simulink model "practica4"  (R2020b)
settings: Solver=ode15s  StartTime=0.0  StopTime=10.0  MaxStep=1E-2  RelTol=1e-3
libraries: fl_lib x10, nesl_utility x6, ee_lib x4, pid_lib x1
settings Model: Creator=demil  LastModifiedBy=demil
settings SolverCC: AlgebraicLoopSolver=LineSearch
settings DataIOCC: SaveFormat=Array  SaveOutput=off  SignalLogging=off  DSMLogging=off  ReturnWorkspaceOutputs=off  TimeSaveName=t
settings DebuggingCC: AlgebraicLoopMsg=none  ArtificialAlgebraicLoopMsg=none  MaxConsecutiveZCsMsg=none  ModelReferenceExtraNoncontSigs=none  OperatingPointInterfaceChecksumMismatchMsg=none

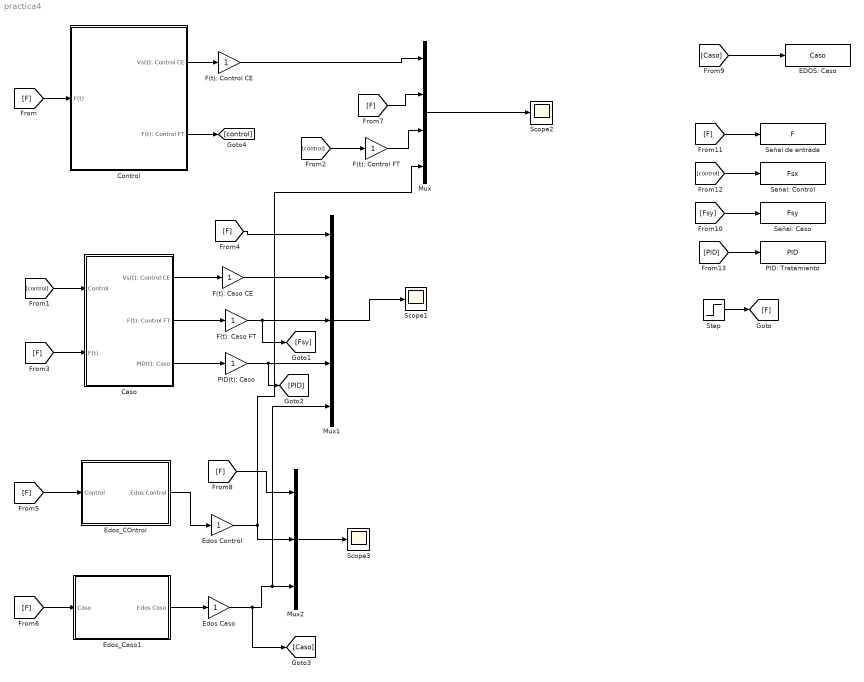
== system practica4 ==
  Caso : Subsystem
  Control : Subsystem
  EDOS: Caso : ToWorkspace  VariableName=Caso  SampleTime=-1
  Edos Caso : Gain
  Edos Control : Gain
  Edos_COntrol : Subsystem
  Edos_Caso1 : Subsystem
  F(t): Caso CE : Gain
  F(t): Caso FT : Gain
  F(t): Control CE : Gain
  F(t): Control FT : Gain
  Mux : Mux
  Mux1 : Mux  Inputs=5
  Mux2 : Mux  Inputs=3
  PID(t): Caso : Gain
  PID: Tratamiento : ToWorkspace  VariableName=PID  SampleTime=-1
  Scope1 : Scope
  Scope2 : Scope
  Scope3 : Scope
  Señal de entrada : ToWorkspace  VariableName=F  SampleTime=-1
  Señal: Caso : ToWorkspace  VariableName=Fsy  SampleTime=-1
  Señal: Control : ToWorkspace  VariableName=Fsx  SampleTime=-1
  Step : Step  Time=0  SampleTime=0
  wires:
  [PID] -> PID: Tratamiento/1
  PID(t): Caso/1 -> Mux1/4, [PID]
  [Fsy] -> Señal: Caso/1
  [control] -> F(t): Control FT/1
  [F] -> Señal de entrada/1
  [F] -> Caso/2(F(t))
  [F] -> Mux1/1
  Mux/1 -> Scope2/1
  F(t): Caso FT/1 -> [Fsy], Mux1/3
  Step/1 -> [F]
  F(t): Caso CE/1 -> Mux1/2
  Control/1(Vs(t): Control CE) -> F(t): Control CE/1
  Mux1/1 -> Scope1/1
  Caso/3(PID(t): Caso) -> PID(t): Caso/1
  [control] -> Caso/1(Control)
  F(t): Control FT/1 -> Mux/3
  [control] -> Señal: Control/1
  [F] -> Control/1(F(t))
  Control/2(F(t): Control FT) -> [control]
  F(t): Control CE/1 -> Mux/1
  Caso/1(Vs(t): Control CE) -> F(t): Caso CE/1
  Caso/2(F(t): Control FT) -> F(t): Caso FT/1
  [F] -> Edos_COntrol/1(Control)
  Edos_COntrol/1(Edos Control) -> Edos Control/1
  Mux2/1 -> Scope3/1
  [F] -> Edos_Caso1/1(Caso)
  Edos_Caso1/1(Edos Caso) -> Edos Caso/1
  Edos Caso/1 -> [Caso], Mux1/5, Mux2/3
  Edos Control/1 -> Mux/4, Mux2/2
  [F] -> Mux2/1
  [F] -> Mux/2
  [Caso] -> EDOS: Caso/1

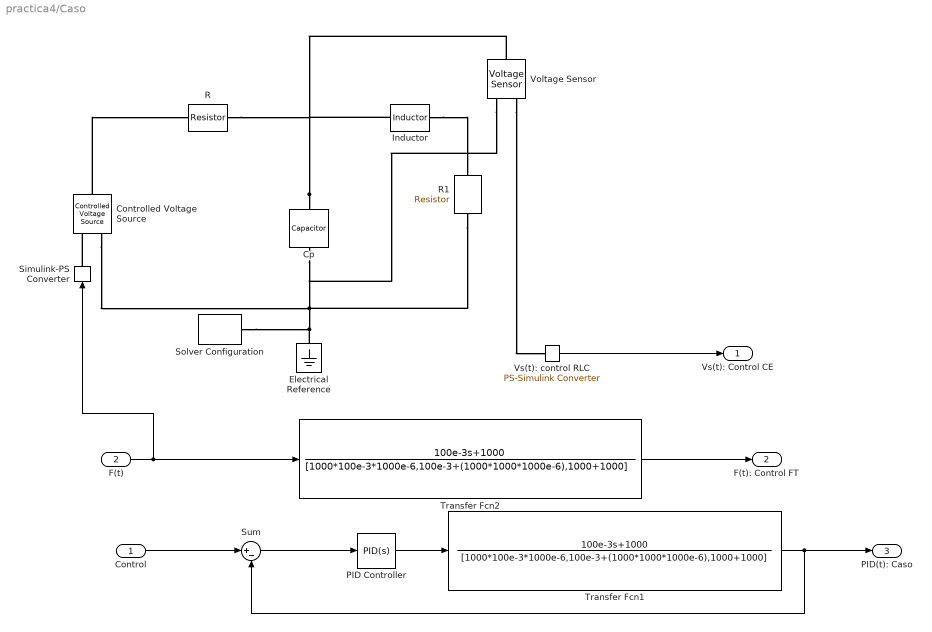
== system practica4/Caso ==
  Control : Inport
  F(t) : Inport  Port=2
  Controlled Voltage Source : fl_lib/Electrical/Electrical Sources/Controlled Voltage Source
  Cp : fl_lib/Electrical/Electrical Elements/Capacitor  c=1000e-6 F  r=1e-6 Ohm  g=0 1/Ohm  i_specify=off  i_priority=None  i=0 A  i_nominal_specify=off  i_nominal_unit=A  i_nominal_value=1  v_specify=off  v_priority=None  v=0 V  v_nominal_specify=off  v_nominal_unit=V  v_nominal_value=1  vc_specify=off  vc_priority=High  vc=0 V  vc_nominal_specify=off  vc_nominal_unit=V  vc_nominal_value=1
  Electrical Reference : fl_lib/Electrical/Electrical Elements/Electrical Reference
  Inductor : fl_lib/Electrical/Electrical Elements/Inductor  l=100e-3 H  r=0 Ohm  g=1e-9 1/Ohm  i_specify=off  i_priority=None  i=0 A  i_nominal_specify=off  i_nominal_unit=A  i_nominal_value=1  v_specify=off  v_priority=None  v=0 V  v_nominal_specify=off  v_nominal_unit=V  v_nominal_value=1  i_L_specify=off  i_L_priority=High  i_L=0 A  i_L_nominal_specify=off  i_L_nominal_unit=A  i_L_nominal_value=1
  PID Controller : pid_lib/PID Controller  Controller=PID  Form=Parallel  TimeDomain=Continuous-time  UseExternalTs=off  SampleTime=-1  IntegratorMethod=Forward Euler  FilterMethod=Forward Euler  ControllerParametersSource=internal  P=665.951561511204  I=82125.2322139515  D=0.178295195912409  UseFilter=on  N=2544.56656071832  TunerSelectOption=Transfer Function Based (PID Tuner App)  InitialConditionSource=internal  InitialConditionForIntegrator=0  InitialConditionForFilter=0  DifferentiatorICPrevScaledInput=0  ExternalReset=none  TrackingMode=off  Kt=1  LimitOutput=off  SatLimitsSource=internal  UpperSaturationLimit=inf  LowerSaturationLimit=-inf  LinearizeAsGain=on  AntiWindupMode=none  Kb=1  POutMin=[]  POutMax=[]  IOutMin=[]  IOutMax=[]  DOutMin=[]  DOutMax=[]  NOutMin=[]  NOutMax=[]  SumOutMin=[]  SumOutMax=[]  SaturationOutMin=[]  SaturationOutMax=[]  PParamMin=[]  PParamMax=[]  IParamMin=[]  IParamMax=[]  DParamMin=[]  DParamMax=[]  NParamMin=[]  NParamMax=[]  KbParamMin=[]  KbParamMax=[]  KtParamMin=[]  KtParamMax=[]  KbOutMin=[]  KbOutMax=[]  KtOutMin=[]  KtOutMax=[]  IntegratorOutMin=[]  IntegratorOutMax=[]  FilterOutMin=[]  FilterOutMax=[]  SumI1OutMin=[]  SumI1OutMax=[]  SumI2OutMin=[]  SumI2OutMax=[]  SumI3OutMin=[]  SumI3OutMax=[]  SumI4OutMin=[]  SumI4OutMax=[]  SumDOutMin=[]  SumDOutMax=[]  DifferentiatorOutMin=[]  DifferentiatorOutMax=[]  FilterDiffOutCoefMin=[]  FilterDiffOutCoefMax=[]  ReciprocalOutMin=[]  ReciprocalOutMax=[]  SumDenOutMin=[]  SumDenOutMax=[]  SumNumOutMin=[]  SumNumOutMax=[]  DivideOutMin=[]  DivideOutMax=[]  UdiffTsProdOutMin=[]  UdiffTsProdOutMax=[]  NTsProdOutMin=[]  NTsProdOutMax=[]  UintegralTsProdOutMin=[]  UintegralTsProdOutMax=[]  UngainTsProdOutMin=[]  UngainTsProdOutMax=[]  IntegratorContinuousStateAttributes=''  IntegratorStateMustResolveToSignalObject=off  IntegratorRTWStateStorageClass=Auto  FilterContinuousStateAttributes=''  FilterStateMustResolveToSignalObject=off  FilterRTWStateStorageClass=Auto  ParallelPVariant=InternalParameters  IdealPVariant=Disabled  IVariant=InternalParameters  DVariant=InternalParameters  IntegratorVariant=Continuous  SatVariant=Disabled  AWVariant=Passthrough  PCopyVariant=Disabled  TRVariant=Disabled  FdbkBlocksVariant=Forward  IdealPFdbkVariant=Disabled  SatFdbkVariant=Disabled  DerivativeFilterVariant=ContFilter  NVariant=InternalParameters  NCopyVariant=Disabled  FilterICVariant=InternalICsFilter  IntegratorICVariant=InternalICs  ExternalResetVariant=Disabled  TRSumVariant=Passthrough  SumFdbkVariant=Disabled  SumVariant=Sum_PID  TsampFilterVariant=InternalTs  TsampNgainVariant=Passthrough  TsampIntegralVariant=Passthrough  ExternalSaturationOutDataTypeStr=Inherit: Same as second input
  R : ee_lib/Passive/Resistor  R=1000 Ohm  R_tol=5  enable_R_tol=0  tol_distribution=1  nSigma=4  enable_operating_limits=0  operating_limit_action=2  max_working_voltage=100 V  power_rating=1 W  enable_faults=0  fault_action=1  R_faulted=inf Ohm  enable_temporal_fault=0  t_fault=1 s  enable_behavioral_fault=0  max_permissible_current=1 A  t_fail_on_current=1 s  noise_mode=0  sample_time=1e-3 s  repeatability=1  auto_seed=2589191353  user_seed=0  Tdevice=25 degC  alpha=3.93e-3 1/K  Tmeas=25 degC  thermal_mass=100 J/K  power_derating_T1=70 degC  power_derating_T2=155 degC  operating_temperature_range_vec=[-50, 150] degC  temperature_specify=off  temperature_priority=High  temperature=298.15 K  temperature_nominal_specify=off  temperature_nominal_unit=K  temperature_nominal_value=1
  R1 : ee_lib/Passive/Resistor  R=1000 Ohm  R_tol=5  enable_R_tol=0  tol_distribution=1  nSigma=4  enable_operating_limits=0  operating_limit_action=2  max_working_voltage=100 V  power_rating=1 W  enable_faults=0  fault_action=1  R_faulted=inf Ohm  enable_temporal_fault=0  t_fault=1 s  enable_behavioral_fault=0  max_permissible_current=1 A  t_fail_on_current=1 s  noise_mode=0  sample_time=1e-3 s  repeatability=1  auto_seed=3054648517  user_seed=0  Tdevice=25 degC  alpha=3.93e-3 1/K  Tmeas=25 degC  thermal_mass=100 J/K  power_derating_T1=70 degC  power_derating_T2=155 degC  operating_temperature_range_vec=[-50, 150] degC  temperature_specify=off  temperature_priority=High  temperature=298.15 K  temperature_nominal_specify=off  temperature_nominal_unit=K  temperature_nominal_value=1
  Simulink-PS Converter : nesl_utility/Simulink-PS Converter  PhysicalDomain=network_engine_domain  SubClassName=ps_input  LeftPortType=input  RightPortType=output  PseudoPeriodic=off  Frequencies=[]  NoiseDistribution=none  NoiseParameters=[]  Unit=1  AffineConversion=off  FilteringAndDerivatives=provide  SimscapeFilterOrder=1  InputFilterTimeConstant=0.001  UdotUserProvided=0
  Solver Configuration : nesl_utility/Solver Configuration  PhysicalDomain=network_engine_domain  SubClassName=solver  LeftPortType=input  RightPortType=generic  Tones=[]  Harmonics=[]  SimulateNoise=off  Profile=off  UseLocalSampling=off  EnableSwitchedLinearOptims=on  FrequencyDomain=off  UseCCode=off  RelTol=0.001  AbsTol=1e-06  MinStep=1e-09  ToWorkspace=off  RevertToSquareIcSolve=off  NumHomotopyIterations=100  PhasorMode=off  PhasorModeNumHarmonics=1  DoDC=off  ResidualTolerance=1e-09  UseLocalSolver=off  LocalSolverChoice=NE_BACKWARD_EULER_ADVANCER  LocalSolverSampleTime=0.001  DoFixedCost=off  MaxNonlinIter=3  MaxModeIter=2  ComputeImpulses=off  ImpulseIterations=2  LinearAlgebra=auto  EquationFormulation=NE_TIME_EF  DelaysMemoryBudget=1024  AutomaticFiltering=on  FilteringTimeConstant=0.001  PartitionStorageMethod=AS_NEEDED  PartitionMemoryBudget=1024  PartitionMethod=ROBUST
  Sum : Sum  Inputs=|+-
  Transfer Fcn1 : TransferFcn  Numerator=[100e-3,1000]  Denominator=[1000*100e-3*1000e-6,100e-3+(1000*1000*1000e-6),1000+1000]
  Transfer Fcn2 : TransferFcn  Numerator=[100e-3,1000]  Denominator=[1000*100e-3*1000e-6,100e-3+(1000*1000*1000e-6),1000+1000]
  Voltage Sensor : fl_lib/Electrical/Electrical Sensors/Voltage Sensor
  "Vs(t): control RLC " : nesl_utility/PS-Simulink Converter  PhysicalDomain=network_engine_domain  SubClassName=ps_output  LeftPortType=input  RightPortType=output  PseudoPeriodic=off  Frequencies=[]  Unit=inherit  AffineConversion=off
  Vs(t): Control CE : Outport
  F(t): Control FT : Outport  Port=2
  PID(t): Caso : Outport  Port=3
  wires:
  Transfer Fcn1/1 -> PID(t): Caso/1, Sum/2
  PID Controller/1 -> Transfer Fcn1/1
  Sum/1 -> PID Controller/1
  Control/1 -> Sum/1
  "Vs(t): control RLC "/1 -> Vs(t): Control CE/1
  F(t)/1 -> Transfer Fcn2/1, Simulink-PS Converter/1
  Transfer Fcn2/1 -> F(t): Control FT/1
  connections:
  Cp/LConn1 -- R/LConn1 -- Voltage Sensor/LConn1 -- Inductor/LConn1
  Solver Configuration/RConn1 -- Voltage Sensor/RConn2 -- Cp/RConn1 -- R1/LConn1 -- Controlled Voltage Source/RConn2 -- Electrical Reference/LConn1
  Voltage Sensor/RConn1 -- "Vs(t): control RLC "/LConn1
  Inductor/RConn1 -- R1/RConn1
  Simulink-PS Converter/RConn1 -- Controlled Voltage Source/RConn1
  Controlled Voltage Source/LConn1 -- R/RConn1

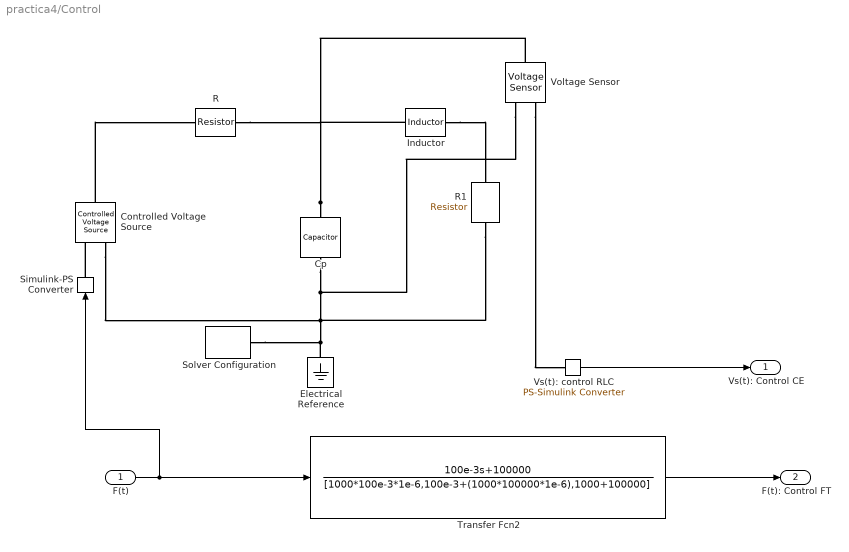
== system practica4/Control ==
  F(t) : Inport
  Controlled Voltage Source : fl_lib/Electrical/Electrical Sources/Controlled Voltage Source
  Cp : fl_lib/Electrical/Electrical Elements/Capacitor  c=1e-6 F  r=1e-6 Ohm  g=0 1/Ohm  i_specify=off  i_priority=None  i=0 A  i_nominal_specify=off  i_nominal_unit=A  i_nominal_value=1  v_specify=off  v_priority=None  v=0 V  v_nominal_specify=off  v_nominal_unit=V  v_nominal_value=1  vc_specify=off  vc_priority=High  vc=0 V  vc_nominal_specify=off  vc_nominal_unit=V  vc_nominal_value=1
  Electrical Reference : fl_lib/Electrical/Electrical Elements/Electrical Reference
  Inductor : fl_lib/Electrical/Electrical Elements/Inductor  l=100e-3 H  r=0 Ohm  g=1e-9 1/Ohm  i_specify=off  i_priority=None  i=0 A  i_nominal_specify=off  i_nominal_unit=A  i_nominal_value=1  v_specify=off  v_priority=None  v=0 V  v_nominal_specify=off  v_nominal_unit=V  v_nominal_value=1  i_L_specify=off  i_L_priority=High  i_L=0 A  i_L_nominal_specify=off  i_L_nominal_unit=A  i_L_nominal_value=1
  R : ee_lib/Passive/Resistor  R=1000 Ohm  R_tol=5  enable_R_tol=0  tol_distribution=1  nSigma=4  enable_operating_limits=0  operating_limit_action=2  max_working_voltage=100 V  power_rating=1 W  enable_faults=0  fault_action=1  R_faulted=inf Ohm  enable_temporal_fault=0  t_fault=1 s  enable_behavioral_fault=0  max_permissible_current=1 A  t_fail_on_current=1 s  noise_mode=0  sample_time=1e-3 s  repeatability=1  auto_seed=2555059182  user_seed=0  Tdevice=25 degC  alpha=3.93e-3 1/K  Tmeas=25 degC  thermal_mass=100 J/K  power_derating_T1=70 degC  power_derating_T2=155 degC  operating_temperature_range_vec=[-50, 150] degC  temperature_specify=off  temperature_priority=High  temperature=298.15 K  temperature_nominal_specify=off  temperature_nominal_unit=K  temperature_nominal_value=1
  R1 : ee_lib/Passive/Resistor  R=100000 Ohm  R_tol=5  enable_R_tol=0  tol_distribution=1  nSigma=4  enable_operating_limits=0  operating_limit_action=2  max_working_voltage=100 V  power_rating=1 W  enable_faults=0  fault_action=1  R_faulted=inf Ohm  enable_temporal_fault=0  t_fault=1 s  enable_behavioral_fault=0  max_permissible_current=1 A  t_fail_on_current=1 s  noise_mode=0  sample_time=1e-3 s  repeatability=1  auto_seed=1126190882  user_seed=0  Tdevice=25 degC  alpha=3.93e-3 1/K  Tmeas=25 degC  thermal_mass=100 J/K  power_derating_T1=70 degC  power_derating_T2=155 degC  operating_temperature_range_vec=[-50, 150] degC  temperature_specify=off  temperature_priority=High  temperature=298.15 K  temperature_nominal_specify=off  temperature_nominal_unit=K  temperature_nominal_value=1
  Simulink-PS Converter : nesl_utility/Simulink-PS Converter  PhysicalDomain=network_engine_domain  SubClassName=ps_input  LeftPortType=input  RightPortType=output  PseudoPeriodic=off  Frequencies=[]  NoiseDistribution=none  NoiseParameters=[]  Unit=1  AffineConversion=off  FilteringAndDerivatives=provide  SimscapeFilterOrder=1  InputFilterTimeConstant=0.001  UdotUserProvided=0
  Solver Configuration : nesl_utility/Solver Configuration  PhysicalDomain=network_engine_domain  SubClassName=solver  LeftPortType=input  RightPortType=generic  Tones=[]  Harmonics=[]  SimulateNoise=off  Profile=off  UseLocalSampling=off  EnableSwitchedLinearOptims=on  FrequencyDomain=off  UseCCode=off  RelTol=0.001  AbsTol=1e-06  MinStep=1e-09  ToWorkspace=off  RevertToSquareIcSolve=off  NumHomotopyIterations=100  PhasorMode=off  PhasorModeNumHarmonics=1  DoDC=off  ResidualTolerance=1e-09  UseLocalSolver=off  LocalSolverChoice=NE_BACKWARD_EULER_ADVANCER  LocalSolverSampleTime=0.001  DoFixedCost=off  MaxNonlinIter=3  MaxModeIter=2  ComputeImpulses=off  ImpulseIterations=2  LinearAlgebra=auto  EquationFormulation=NE_TIME_EF  DelaysMemoryBudget=1024  AutomaticFiltering=on  FilteringTimeConstant=0.001  PartitionStorageMethod=AS_NEEDED  PartitionMemoryBudget=1024  PartitionMethod=ROBUST
  Transfer Fcn2 : TransferFcn  Numerator=[100e-3,100000]  Denominator=[1000*100e-3*1e-6,100e-3+(1000*100000*1e-6),1000+100000]
  Voltage Sensor : fl_lib/Electrical/Electrical Sensors/Voltage Sensor
  "Vs(t): control RLC " : nesl_utility/PS-Simulink Converter  PhysicalDomain=network_engine_domain  SubClassName=ps_output  LeftPortType=input  RightPortType=output  PseudoPeriodic=off  Frequencies=[]  Unit=inherit  AffineConversion=off
  Vs(t): Control CE : Outport
  F(t): Control FT : Outport  Port=2
  wires:
  Transfer Fcn2/1 -> F(t): Control FT/1
  F(t)/1 -> Transfer Fcn2/1, Simulink-PS Converter/1
  "Vs(t): control RLC "/1 -> Vs(t): Control CE/1
  connections:
  Cp/RConn1 -- Electrical Reference/LConn1 -- Solver Configuration/RConn1 -- R1/LConn1 -- Controlled Voltage Source/RConn2 -- Voltage Sensor/RConn2
  Cp/LConn1 -- R/LConn1 -- Voltage Sensor/LConn1 -- Inductor/LConn1
  Voltage Sensor/RConn1 -- "Vs(t): control RLC "/LConn1
  Inductor/RConn1 -- R1/RConn1
  Controlled Voltage Source/LConn1 -- R/RConn1
  Simulink-PS Converter/RConn1 -- Controlled Voltage Source/RConn1

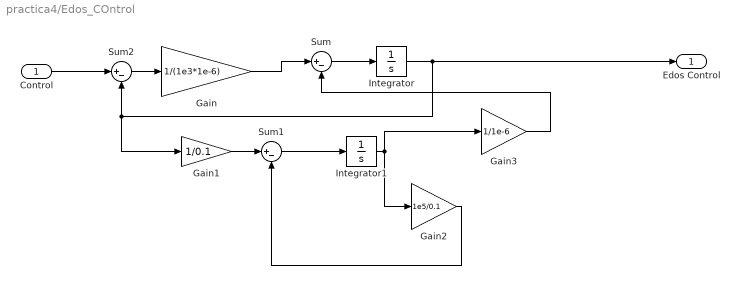
== system practica4/Edos_COntrol ==
  Control : Inport
  Gain : Gain  Gain=1/(1e3*1e-6)
  Gain1 : Gain  Gain=1/0.1
  Gain2 : Gain  Gain=1e5/0.1
  Gain3 : Gain  Gain=1/1e-6
  Integrator : Integrator
  Integrator1 : Integrator
  Sum : Sum  Inputs=|+-
  Sum1 : Sum  Inputs=|+-
  Sum2 : Sum  Inputs=|+-
  Edos Control : Outport
  wires:
  Control/1 -> Sum2/1
  Sum2/1 -> Gain/1
  Gain/1 -> Sum/1
  Sum/1 -> Integrator/1
  Integrator/1 -> Sum2/2, Gain1/1, Edos Control/1
  Gain1/1 -> Sum1/1
  Sum1/1 -> Integrator1/1
  Integrator1/1 -> Gain3/1, Gain2/1
  Gain2/1 -> Sum1/2
  Gain3/1 -> Sum/2

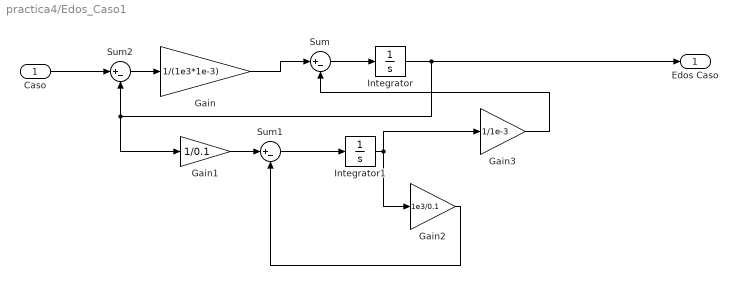
== system practica4/Edos_Caso1 ==
  Caso : Inport
  Gain : Gain  Gain=1/(1e3*1e-3)
  Gain1 : Gain  Gain=1/0.1
  Gain2 : Gain  Gain=1e3/0.1
  Gain3 : Gain  Gain=1/1e-3
  Integrator : Integrator
  Integrator1 : Integrator
  Sum : Sum  Inputs=|+-
  Sum1 : Sum  Inputs=|+-
  Sum2 : Sum  Inputs=|+-
  Edos Caso : Outport
  wires:
  Caso/1 -> Sum2/1
  Sum2/1 -> Gain/1
  Gain/1 -> Sum/1
  Sum/1 -> Integrator/1
  Integrator/1 -> Sum2/2, Gain1/1, Edos Caso/1
  Gain1/1 -> Sum1/1
  Sum1/1 -> Integrator1/1
  Integrator1/1 -> Gain3/1, Gain2/1
  Gain2/1 -> Sum1/2
  Gain3/1 -> Sum/2
